simulink model "Me492CasterM0"  (R2026b)
settings: Solver=ode4  StopTime=4  FixedStep=solver_step_s
model workspace (MAT data in the model file):
  body_origin = 'drive_axle_midpoint_projected_to_ground'
  caster_pivot_m = [-0.18; 0; 0.1]
  caster_pivot_x_m = -0.18
  caster_pivot_y_m = 0
  caster_radius_m = 0.04
  caster_trail_m = 0.05
  caster_width_m = 0.02
  chassis_center_m = [0; 0; 0.14]
  chassis_size_m = [0.5; 0.32; 0.08]
  command_array = [0 0.02 0.04 0.06 0.08 0.1 0.12 0.14 0.16 0.18 0.2 0.22 ... (603 elements, 201x3)]
  command_sample_dt_s = 0.02
  drive_radius_m = 0.075
  drive_track_m = 0.38
  drive_width_m = 0.03
  fork_plate_thickness_m = 0.006
  fork_stem_radius_m = 0.008
  fork_yoke_gap_m = 0.026
  initial_caster_angle_rad = 0
  initial_x_m = 0
  initial_y_m = 0
  initial_yaw_rad = 0
  parameter_status = 'provisional_synthetic'
  schema_version = 'me492-caster-v0.1'
  solver_step_s = 0.001
  units = 'SI'
settings Model: Creator=lelfs  LastModifiedBy=lelfs
settings DataIOCC: SaveOutput=off  SignalLogging=off

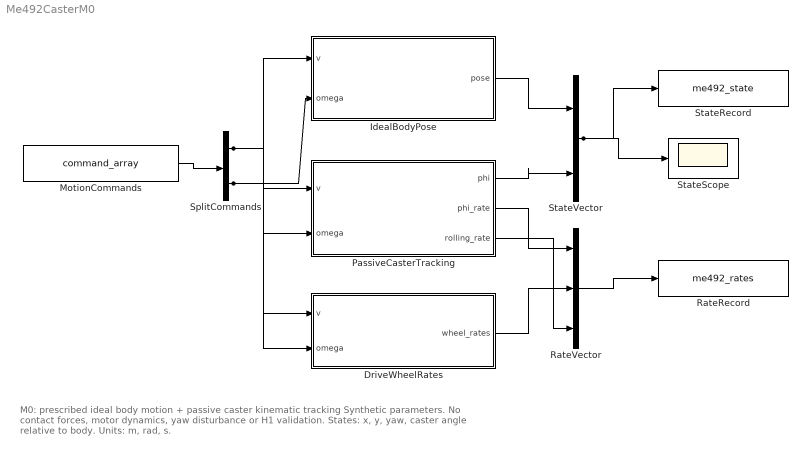
== system Me492CasterM0 ==
  note: M0: prescribed ideal body motion + passive caster kinematic tracking
      | Synthetic parameters. No contact forces, motor dynamics, yaw disturbance or H1 validation.
      | States: x, y, yaw, caster angle relative to body. Units: m, rad, s.
  DriveWheelRates : Subsystem
  IdealBodyPose : Subsystem
  MotionCommands : FromWorkspace  VariableName=command_array  SampleTime=command_sample_dt_s  Interpolate=off  OutputAfterFinalValue=Holding final value
  PassiveCasterTracking : Subsystem
  RateRecord : ToWorkspace  VariableName=me492_rates  SaveFormat=Timeseries  SampleTime=-1
  RateVector : Mux  Inputs=3
  SplitCommands : Demux  Outputs=2
  StateRecord : ToWorkspace  VariableName=me492_state  SaveFormat=Timeseries  SampleTime=-1
  StateScope : Scope
  StateVector : Mux  Inputs=2
  wires:
  MotionCommands/1 -> SplitCommands/1
  SplitCommands/1 -> IdealBodyPose/1(v), PassiveCasterTracking/1(v), DriveWheelRates/1(v)
  SplitCommands/2 -> IdealBodyPose/2(omega), PassiveCasterTracking/2(omega), DriveWheelRates/2(omega)
  IdealBodyPose/1(pose) -> StateVector/1
  PassiveCasterTracking/1(phi) -> StateVector/2
  PassiveCasterTracking/2(phi_rate) -> RateVector/1
  DriveWheelRates/1(wheel_rates) -> RateVector/2
  PassiveCasterTracking/3(rolling_rate) -> RateVector/3
  StateVector/1 -> StateRecord/1, StateScope/1
  RateVector/1 -> RateRecord/1

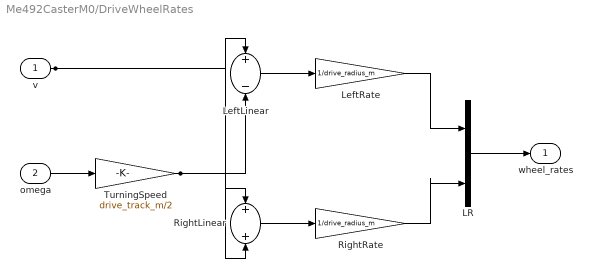
== system Me492CasterM0/DriveWheelRates ==
  v : Inport
  omega : Inport  Port=2
  LR : Mux  Inputs=2
  LeftLinear : Sum  Inputs=+-
  LeftRate : Gain  Gain=1/drive_radius_m
  RightLinear : Sum
  RightRate : Gain  Gain=1/drive_radius_m
  TurningSpeed : Gain  Gain=drive_track_m/2
  wheel_rates : Outport
  wires:
  omega/1 -> TurningSpeed/1
  v/1 -> LeftLinear/1, RightLinear/1
  TurningSpeed/1 -> LeftLinear/2, RightLinear/2
  LeftLinear/1 -> LeftRate/1
  RightLinear/1 -> RightRate/1
  LeftRate/1 -> LR/1
  RightRate/1 -> LR/2
  LR/1 -> wheel_rates/1

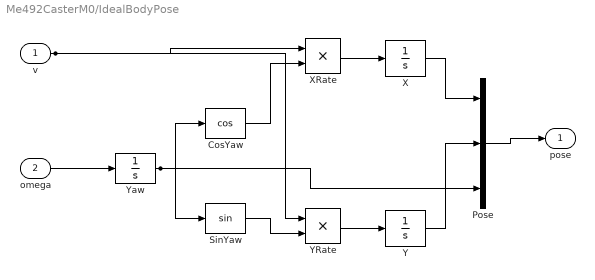
== system Me492CasterM0/IdealBodyPose ==
  v : Inport
  omega : Inport  Port=2
  CosYaw : Trigonometry  Operator=cos
  Pose : Mux  Inputs=3
  SinYaw : Trigonometry
  X : Integrator  InitialCondition=initial_x_m
  XRate : Product
  Y : Integrator  InitialCondition=initial_y_m
  YRate : Product
  Yaw : Integrator  InitialCondition=initial_yaw_rad
  pose : Outport
  wires:
  omega/1 -> Yaw/1
  Yaw/1 -> CosYaw/1, SinYaw/1, Pose/3
  v/1 -> XRate/1, YRate/1
  CosYaw/1 -> XRate/2
  XRate/1 -> X/1
  SinYaw/1 -> YRate/2
  YRate/1 -> Y/1
  X/1 -> Pose/1
  Y/1 -> Pose/2
  Pose/1 -> pose/1

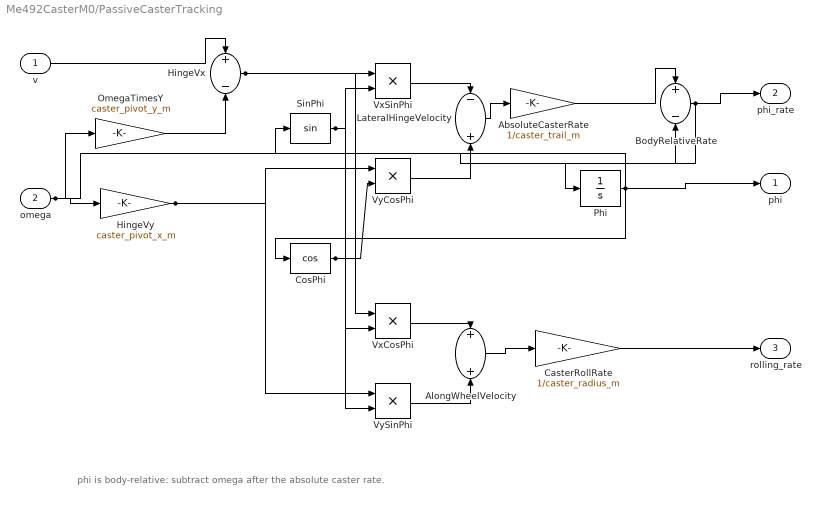
== system Me492CasterM0/PassiveCasterTracking ==
  note: phi is body-relative: subtract omega after the absolute caster rate.
  v : Inport
  omega : Inport  Port=2
  AbsoluteCasterRate : Gain  Gain=1/caster_trail_m
  AlongWheelVelocity : Sum
  BodyRelativeRate : Sum  Inputs=+-
  CasterRollRate : Gain  Gain=1/caster_radius_m
  CosPhi : Trigonometry  Operator=cos
  HingeVx : Sum  Inputs=+-
  HingeVy : Gain  Gain=caster_pivot_x_m
  LateralHingeVelocity : Sum  Inputs=-+
  OmegaTimesY : Gain  Gain=caster_pivot_y_m
  Phi : Integrator  InitialCondition=initial_caster_angle_rad
  SinPhi : Trigonometry
  VxCosPhi : Product
  VxSinPhi : Product
  VyCosPhi : Product
  VySinPhi : Product
  phi : Outport
  phi_rate : Outport  Port=2
  rolling_rate : Outport  Port=3
  wires:
  omega/1 -> OmegaTimesY/1, HingeVy/1, BodyRelativeRate/2
  v/1 -> HingeVx/1
  OmegaTimesY/1 -> HingeVx/2
  Phi/1 -> SinPhi/1, CosPhi/1, phi/1
  HingeVx/1 -> VxSinPhi/1, VxCosPhi/1
  SinPhi/1 -> VxSinPhi/2, VySinPhi/2
  HingeVy/1 -> VyCosPhi/1, VySinPhi/1
  CosPhi/1 -> VyCosPhi/2, VxCosPhi/2
  VxSinPhi/1 -> LateralHingeVelocity/1
  VyCosPhi/1 -> LateralHingeVelocity/2
  LateralHingeVelocity/1 -> AbsoluteCasterRate/1
  AbsoluteCasterRate/1 -> BodyRelativeRate/1
  BodyRelativeRate/1 -> Phi/1, phi_rate/1
  VxCosPhi/1 -> AlongWheelVelocity/1
  VySinPhi/1 -> AlongWheelVelocity/2
  AlongWheelVelocity/1 -> CasterRollRate/1
  CasterRollRate/1 -> rolling_rate/1
